simulink model "plantaCPC_2025"  (R2025b)
settings: Solver=ode4  StartTime=0.0  StopTime=50  RelTol=1e-3  EnableMultiTasking=on
values from neighbouring files (symbols this model uses):
  A = 0.159    [Fuzzy_no_anfis_sim.m]    (also in build_FLC_L4_anfis.m = zeros(size(Xtr,1), nOut); build_FLC_lower_single.m; build_FLC_upper_single.m; fuzzym.m)
  a1 = 6.1360e-04    (= 0.0006136)    [Fuzzy_no_anfis_sim.m]    (also in build_FLC_lower_single.m; fuzzym.m)
  a2 = 5.4678e-04    (= 0.00054678)    [Fuzzy_no_anfis_sim.m]    (also in build_FLC_lower_single.m; fuzzym.m)
  a3 = 3.5752e-04    (= 0.00035752)    [Fuzzy_no_anfis_sim.m]    (also in build_FLC_lower_single.m; fuzzym.m)
  a4 = 4.1820e-04    (= 0.0004182)    [Fuzzy_no_anfis_sim.m]    (also in build_FLC_L4_anfis.m; build_FLC_L4_single.m; build_FLC_lower_single.m; fuzzym.m)
  gamma1 = 0.455    [Fuzzy_no_anfis_sim.m]    (also in build_FLC_L4_anfis.m; build_FLC_L4_single.m; build_FLC_lower_single.m; fuzzym.m)
  gamma2 = 0.4195    [Fuzzy_no_anfis_sim.m]    (also in build_FLC_lower_single.m; fuzzym.m)
  k1 = q_max    (= 0.0017)    [Fuzzy_no_anfis_sim.m]    (also in build_FLC_L4_anfis.m; build_FLC_L4_single.m; fuzzym.m)
  k2 = q_max    (= 0.0017)    [Fuzzy_no_anfis_sim.m]    (also in fuzzym.m)
libraries: simulink x16, fuzblock x1
settings Model: Creator=Administrator  LastModifiedBy=wepi
settings SolverCC: AlgebraicLoopSolver=TrustRegion
settings DataIOCC: LimitDataPoints=on  SaveFormat=Array  ReturnWorkspaceOutputs=off
settings OptimizationCC: LifeSpan=inf
settings DebuggingCC: UnderspecifiedInitializationDetection=Classic  MergeDetectMultiDrivingBlocksExec=none  SolverPrmCheckMsg=warning  UnconnectedInputMsg=warning  UnconnectedOutputMsg=warning  UnconnectedLineMsg=warning  StateNameClashWarn=warning  SFUnexpectedBacktrackingDiag=warning  SFNoUnconditionalDefaultTransitionDiag=warning  SFExecutionAtInitializationDiag=none  ArithmeticOperatorsInVariantConditions=warning
settings HardwareCC: ProdBitPerPointer=32.0  ProdBitPerSizeT=32.0  ProdBitPerPtrDiffT=32.0  ProdLargestAtomicFloat=None  ProdIntDivRoundTo=Undefined  ProdEndianess=Unspecified  ProdWordSize=32.0  ProdHWDeviceType=32-bit Generic
settings ModelReferenceCC: PropagateSignalLabelsOutOfModel=off
settings SFSimCC: SimUseLocalCustomCode=off  CustomCodeUndefinedFunction=UseInterfaceOnly
settings RTWCC: RTWUseLocalCustomCode=off  GPUComputeCapability=3.5
settings CodeAppCC: StateflowObjectComments=on
settings GRTTargetCC: TargetLangStandard=C89/C90 (ANSI)
settings ConfigComp: CovMetricSettings=dw  CovSaveCumulativeToWorkspaceVar=on  CovSaveSingleToWorkspaceVar=on  CovExternalEMLEnable=off

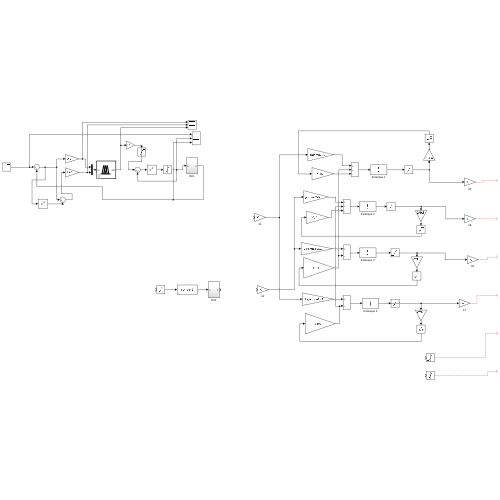
[thumbnail: Simulink's stored preview of the top-level diagram]
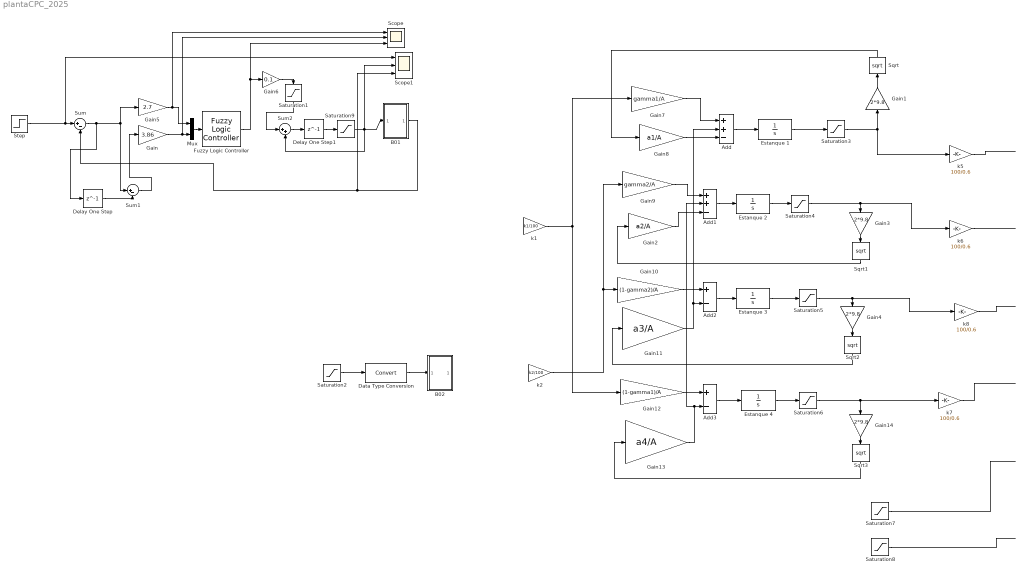
== system plantaCPC_2025 ==
  Add : Sum  Inputs=++-
  Add1 : Sum  Inputs=++-
  Add2 : Sum  Inputs=+-
  Add3 : Sum  Inputs=+-
  B01 : Subsystem
  B02 : Subsystem
  Data Type Conversion : DataTypeConversion  SaturateOnIntegerOverflow=off  RndMeth=Floor
  Delay One Step : Delay  DelayLength=1  SampleTime=0.1
  Delay One Step1 : Delay  DelayLength=1  SampleTime=0.1
  Estanque 1 : TransferFcn  Denominator=[1 0]
  "Estanque 2 " : TransferFcn  Denominator=[1 0]
  Estanque 3 : TransferFcn  Denominator=[1 0]
  Estanque 4 : TransferFcn  Denominator=[1 0]
  Fuzzy Logic Controller : fuzblock/Fuzzy Logic  Controller  FIS=fis  OutputSampleNumber=101  DataType=double  UseLookupTable=off  NumBreakpoints=10  FuzzifiedInputs=off  RuleFiringStrengths=off  RuleOutputs=off  AggregatedOutputs=off  SimulateUsing=Interpreted execution  OutOfRangeInputValueMessage=warning  NoRuleFiredMessage=warning  EmptyOutputFuzzySetMessage=warning
  Gain : Gain  Gain=3.86
  Gain{1,3..4,14} (4 alike) : Gain  Gain=2*9.8
  Gain10 : Gain  Gain=(1-gamma2)/A
  Gain11 : Gain  Gain=a3/A
  Gain12 : Gain  Gain=(1-gamma1)/A
  Gain13 : Gain  Gain=a4/A
  Gain2 : Gain  Gain=a2/A
  Gain5 : Gain  Gain=2.7
  Gain6 : Gain  Gain=0.1
  Gain7 : Gain  Gain=gamma1/A
  Gain8 : Gain  Gain=a1/A
  Gain9 : Gain  Gain=gamma2/A
  Mux : Mux  Inputs=2
  Saturation1 : Saturate  UpperLimit=100  LowerLimit=-100
  Saturation{2,7..9} (4 alike) : Saturate  UpperLimit=100  LowerLimit=0
  Saturation{3..6} (4 alike) : Saturate  UpperLimit=0.8  LowerLimit=0
  Scope : Scope  NumInputPorts=3
      settings: ActiveDisplayYMinimum=103.80137956396959  ActiveDisplayYMaximum=139.96234120398589
  Scope1 : Scope  NumInputPorts=3
      settings: ActiveDisplayYMinimum=-31.330783914246943  ActiveDisplayYMaximum=99.163140980507663
  Sqrt{,1..3} (4 alike) : Sqrt
  Step : Step  Time=30  Before=40  After=50  SampleTime=0
  Sum : Sum  Inputs=|+-
  Sum1 : Sum  Inputs=|+-
  Sum2 : Sum  Inputs=|++
  k1 : Gain  Gain=k1/100
  k2 : Gain  Gain=k2/100
  k{5..8} (4 alike) : Gain  Gain=100/0.6
  wires:
  Saturation3/1 -> k5/1, Gain1/1
  Saturation4/1 -> k6/1, Gain3/1
  Saturation5/1 -> k8/1, Gain4/1
  Estanque 1/1 -> Saturation3/1
  "Estanque 2 "/1 -> Saturation4/1
  Estanque 4/1 -> Saturation6/1
  Saturation2/1 -> Data Type Conversion/1
  Fuzzy Logic Controller/1 -> Gain6/1, Scope/3
  Gain7/1 -> Add/1
  k1/1 -> Gain12/1, Gain7/1
  Gain8/1 -> Add/3
  Add/1 -> Estanque 1/1
  Add1/1 -> "Estanque 2 "/1
  Add2/1 -> Estanque 3/1
  Add3/1 -> Estanque 4/1
  Gain9/1 -> Add1/1
  k2/1 -> Gain9/1, Gain10/1
  Gain2/1 -> Add1/3
  Gain10/1 -> Add2/1
  Gain11/1 -> Add/2, Add2/2
  Gain12/1 -> Add3/1
  Gain13/1 -> Add1/2, Add3/2
  Estanque 3/1 -> Saturation5/1
  Gain1/1 -> Sqrt/1
  Sqrt/1 -> Gain8/1
  Gain3/1 -> Sqrt1/1
  Sqrt1/1 -> Gain2/1
  Gain4/1 -> Sqrt2/1
  Gain14/1 -> Sqrt3/1
  Saturation6/1 -> Gain14/1, k7/1
  Sqrt3/1 -> Gain13/1
  Sqrt2/1 -> Gain11/1
  Data Type Conversion/1 -> B02/1(In1)
  Sum2/1 -> Delay One Step1/1
  Saturation7/1 -> ?
  Saturation8/1 -> ?
  k8/1 -> ?
  k6/1 -> ?
  k5/1 -> ?
  k7/1 -> ?
  Sum/1 -> Gain5/1, Sum1/1, Delay One Step/1
  Step/1 -> Scope1/1, Sum/1
  Mux/1 -> Fuzzy Logic Controller/1
  Delay One Step/1 -> Sum1/2
  Sum1/1 -> Gain/1
  Gain/1 -> Scope/2, Mux/2
  Gain5/1 -> Scope/1, Mux/1
  Saturation9/1 -> Sum2/2, Scope1/2, B01/1(In1)
  Delay One Step1/1 -> Saturation9/1
  B01/1(Out1) -> Sum/2, Scope1/3
  Gain6/1 -> Saturation1/1
  Saturation1/1 -> Sum2/1

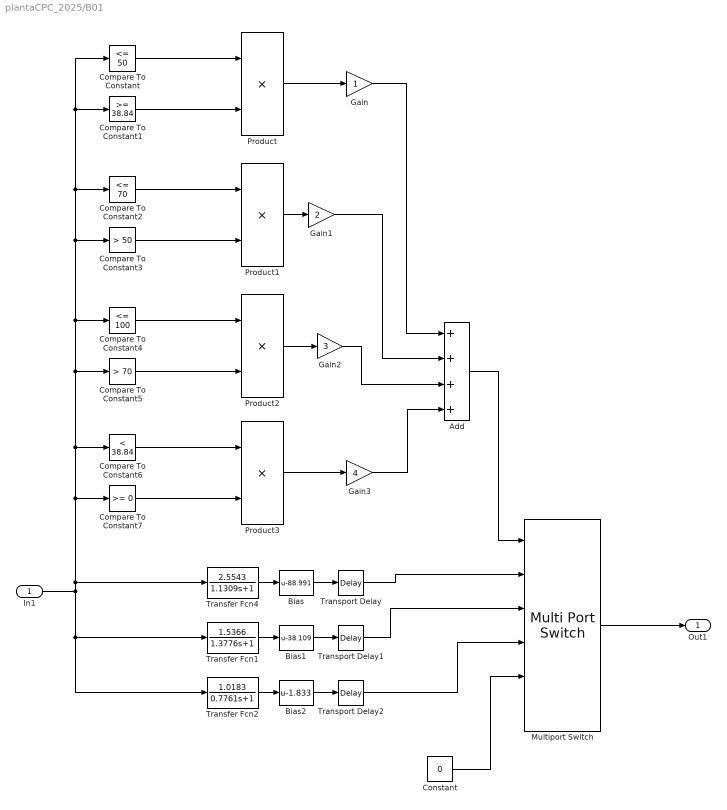
== system plantaCPC_2025/B01 ==
  In1 : Inport
  Add : Sum  Inputs=++++
  Bias : Bias  Bias=-88.991  SaturateOnIntegerOverflow=off
  Bias1 : Bias  Bias=-38.109  SaturateOnIntegerOverflow=off
  Bias2 : Bias  Bias=-1.833  SaturateOnIntegerOverflow=off
  Compare To Constant : simulink/Logic and Bit Operations/Compare To Constant  relop=<=  const=50  OutDataTypeStr=boolean
  Compare To Constant1 : simulink/Logic and Bit Operations/Compare To Constant  relop=>=  const=38.84  OutDataTypeStr=boolean
  Compare To Constant2 : simulink/Logic and Bit Operations/Compare To Constant  relop=<=  const=70  OutDataTypeStr=boolean
  Compare To Constant3 : simulink/Logic and Bit Operations/Compare To Constant  relop=>  const=50  OutDataTypeStr=boolean
  Compare To Constant4 : simulink/Logic and Bit Operations/Compare To Constant  relop=<=  const=100  OutDataTypeStr=boolean
  Compare To Constant5 : simulink/Logic and Bit Operations/Compare To Constant  relop=>  const=70  OutDataTypeStr=boolean
  Compare To Constant6 : simulink/Logic and Bit Operations/Compare To Constant  relop=<  const=38.84  OutDataTypeStr=boolean
  Compare To Constant7 : simulink/Logic and Bit Operations/Compare To Constant  relop=>=  const=0  OutDataTypeStr=boolean
  Constant : Constant  Value=0
  Gain : Gain
  Gain1 : Gain  Gain=2
  Gain2 : Gain  Gain=3
  Gain3 : Gain  Gain=4
  Multiport Switch : MultiPortSwitch  Inputs=5  SaturateOnIntegerOverflow=off  InputSameDT=off
  Product{,1..3} (4 alike) : Product
  Transfer Fcn1 : TransferFcn  Numerator=[1.5366]  Denominator=[1.3776 1]
  Transfer Fcn2 : TransferFcn  Numerator=[1.0183]  Denominator=[0.7761 1]
  Transfer Fcn4 : TransferFcn  Numerator=[2.5543]  Denominator=[1.1309 1]
  Transport Delay : TransportDelay  DelayTime=0.6
  Transport Delay1 : TransportDelay  DelayTime=0.5
  Transport Delay2 : TransportDelay  DelayTime=0.5
  Out1 : Outport
  wires:
  Multiport Switch/1 -> Out1/1
  Product/1 -> Gain/1
  Gain/1 -> Add/1
  Product1/1 -> Gain1/1
  Gain1/1 -> Add/2
  Gain2/1 -> Add/3
  Product2/1 -> Gain2/1
  Add/1 -> Multiport Switch/1
  Compare To Constant/1 -> Product/1
  Transfer Fcn4/1 -> Bias/1
  Transfer Fcn1/1 -> Bias1/1
  Transfer Fcn2/1 -> Bias2/1
  Compare To Constant1/1 -> Product/2
  Compare To Constant2/1 -> Product1/1
  Compare To Constant3/1 -> Product1/2
  Compare To Constant4/1 -> Product2/1
  Compare To Constant5/1 -> Product2/2
  Transport Delay1/1 -> Multiport Switch/3
  Transport Delay2/1 -> Multiport Switch/4
  Bias/1 -> Transport Delay/1
  Bias1/1 -> Transport Delay1/1
  Bias2/1 -> Transport Delay2/1
  Product3/1 -> Gain3/1
  Compare To Constant6/1 -> Product3/1
  Compare To Constant7/1 -> Product3/2
  In1/1 -> Compare To Constant7/1, Compare To Constant6/1, Compare To Constant4/1, Compare To Constant2/1, Compare To Constant1/1, Compare To Constant/1, Compare To Constant3/1, Compare To Constant5/1, Transfer Fcn4/1, Transfer Fcn2/1, Transfer Fcn1/1
  Gain3/1 -> Add/4
  Constant/1 -> Multiport Switch/5
  Transport Delay/1 -> Multiport Switch/2

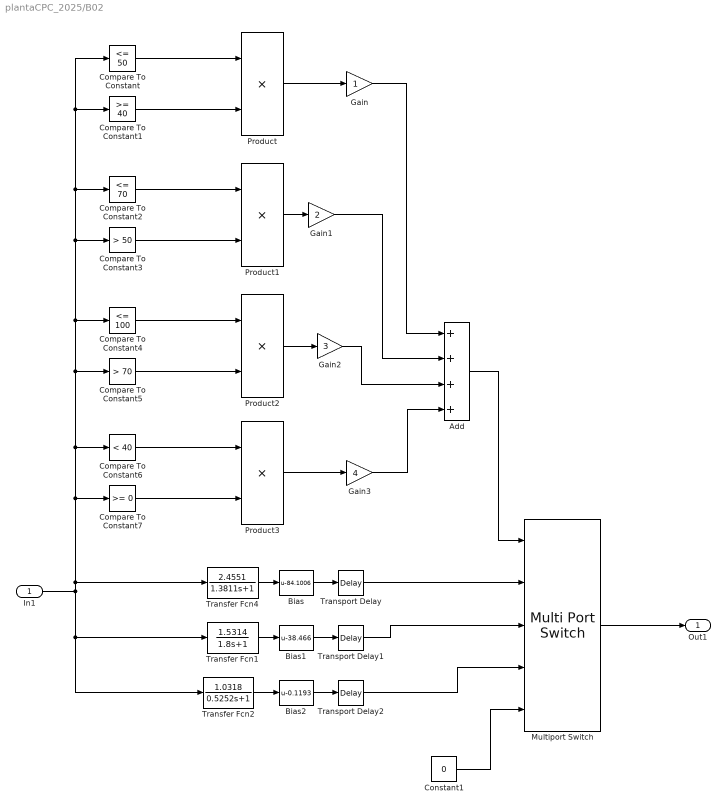
== system plantaCPC_2025/B02 ==
  In1 : Inport
  Add : Sum  Inputs=++++
  Bias : Bias  Bias=-84.1006  SaturateOnIntegerOverflow=off
  Bias1 : Bias  Bias=-38.466  SaturateOnIntegerOverflow=off
  Bias2 : Bias  Bias=-0.1193  SaturateOnIntegerOverflow=off
  Compare To Constant : simulink/Logic and Bit Operations/Compare To Constant  relop=<=  const=50  OutDataTypeStr=boolean
  Compare To Constant1 : simulink/Logic and Bit Operations/Compare To Constant  relop=>=  const=40  OutDataTypeStr=boolean
  Compare To Constant2 : simulink/Logic and Bit Operations/Compare To Constant  relop=<=  const=70  OutDataTypeStr=boolean
  Compare To Constant3 : simulink/Logic and Bit Operations/Compare To Constant  relop=>  const=50  OutDataTypeStr=boolean
  Compare To Constant4 : simulink/Logic and Bit Operations/Compare To Constant  relop=<=  const=100  OutDataTypeStr=boolean
  Compare To Constant5 : simulink/Logic and Bit Operations/Compare To Constant  relop=>  const=70  OutDataTypeStr=boolean
  Compare To Constant6 : simulink/Logic and Bit Operations/Compare To Constant  relop=<  const=40  OutDataTypeStr=boolean
  Compare To Constant7 : simulink/Logic and Bit Operations/Compare To Constant  relop=>=  const=0  OutDataTypeStr=boolean
  Constant1 : Constant  Value=0
  Gain : Gain
  Gain1 : Gain  Gain=2
  Gain2 : Gain  Gain=3
  Gain3 : Gain  Gain=4
  Multiport Switch : MultiPortSwitch  Inputs=4  SaturateOnIntegerOverflow=off  InputSameDT=off
  Product{,1..3} (4 alike) : Product
  Transfer Fcn1 : TransferFcn  Numerator=[1.5314]  Denominator=[1.8 1]
  Transfer Fcn2 : TransferFcn  Numerator=[1.0318]  Denominator=[0.5252 1]
  Transfer Fcn4 : TransferFcn  Numerator=[2.4551]  Denominator=[1.3811 1]
  Transport Delay : TransportDelay  DelayTime=0.5
  Transport Delay1 : TransportDelay  DelayTime=0.5
  Transport Delay2 : TransportDelay  DelayTime=0.8
  Out1 : Outport
  wires:
  Multiport Switch/1 -> Out1/1
  Product/1 -> Gain/1
  Gain/1 -> Add/1
  Product1/1 -> Gain1/1
  Gain1/1 -> Add/2
  Gain2/1 -> Add/3
  Product2/1 -> Gain2/1
  Add/1 -> Multiport Switch/1
  Compare To Constant/1 -> Product/1
  Transfer Fcn4/1 -> Bias/1
  Transfer Fcn1/1 -> Bias1/1
  Transfer Fcn2/1 -> Bias2/1
  Compare To Constant1/1 -> Product/2
  Compare To Constant2/1 -> Product1/1
  Compare To Constant3/1 -> Product1/2
  Compare To Constant4/1 -> Product2/1
  Compare To Constant5/1 -> Product2/2
  Transport Delay/1 -> Multiport Switch/2
  Transport Delay1/1 -> Multiport Switch/3
  Transport Delay2/1 -> Multiport Switch/4
  Bias/1 -> Transport Delay/1
  Bias1/1 -> Transport Delay1/1
  Bias2/1 -> Transport Delay2/1
  Product3/1 -> Gain3/1
  Compare To Constant6/1 -> Product3/1
  Compare To Constant7/1 -> Product3/2
  In1/1 -> Compare To Constant7/1, Compare To Constant6/1, Compare To Constant4/1, Compare To Constant2/1, Compare To Constant1/1, Compare To Constant/1, Compare To Constant3/1, Compare To Constant5/1, Transfer Fcn4/1, Transfer Fcn2/1, Transfer Fcn1/1
  Gain3/1 -> Add/4
  Constant1/1 -> Multiport Switch/5
